simulink model "adaptive_joint_space_control"  (R2024b)
settings: Solver=VariableStepAuto  StartTime=0.0  StopTime=24*5  RelTol=1e-3
undefined symbols (not defined in the file): DiscIntNeverNeededParam, K_pi, Kd_c_ad, lambda, ml, pi0, q0, Tc
settings Model: Creator=storm  LastModifiedBy=giaco
settings OptimizationCC: ReuseModelBlockBuffer=off
settings DebuggingCC: UnconnectedInputMsg=warning  UnconnectedOutputMsg=warning  UnconnectedLineMsg=warning
settings ModelReferenceCC: EnableRefExpFcnMdlSchedulingChecks=on
settings RTWCC: GPUComputeCapability=3.5  DLArmComputeVersion=19.05

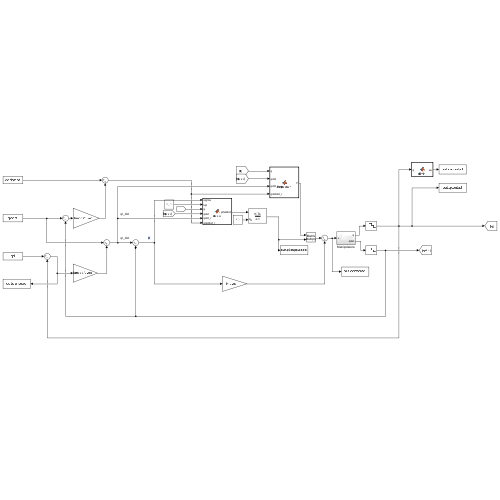
[thumbnail: Simulink's stored preview of the top-level diagram]
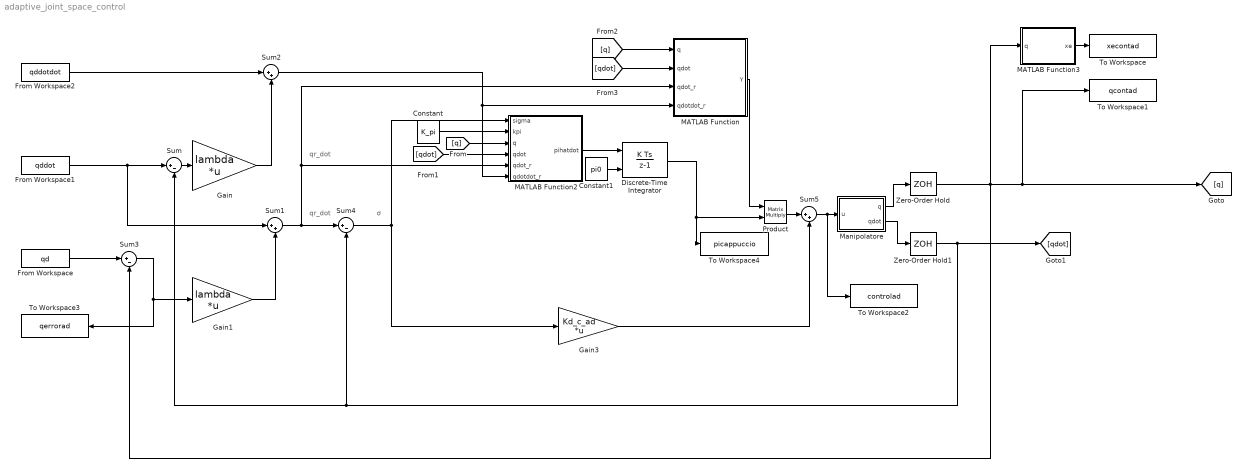
== system adaptive_joint_space_control ==
  note: σ
  note: qr_dot
  note: qr_dot
  Constant : Constant  Value=K_pi
  Constant1 : Constant  Value=pi0
  Discrete-Time Integrator : DiscreteIntegrator  InitialConditionSource=external  SampleTime=Tc  ICPrevOutput=DiscIntNeverNeededParam  ICPrevScaledInput=DiscIntNeverNeededParam
  From Workspace : FromWorkspace  VariableName=qd  SampleTime=Tc
  From Workspace1 : FromWorkspace  VariableName=qddot  SampleTime=Tc
  From Workspace2 : FromWorkspace  VariableName=qddotdot  SampleTime=Tc
  Gain : Gain  Gain=lambda  Multiplication=Matrix(K*u) (u vector)
  Gain1 : Gain  Gain=lambda  Multiplication=Matrix(K*u) (u vector)
  Gain3 : Gain  Gain=Kd_c_ad  Multiplication=Matrix(K*u) (u vector)
  MATLAB Function : MATLAB Function  TreatAsAtomicUnit=on
  MATLAB Function2 : MATLAB Function  TreatAsAtomicUnit=on
  MATLAB Function3 : MATLAB Function  TreatAsAtomicUnit=on
  Manipolatore : Subsystem
  Product : Product  Multiplication=Matrix(*)
  Sum : Sum  Inputs=|+-
  Sum1 : Sum  Inputs=|++
  Sum2 : Sum  Inputs=|++
  Sum3 : Sum  Inputs=|+-
  Sum4 : Sum  Inputs=|+-
  Sum5 : Sum  Inputs=|++
  To Workspace : ToWorkspace  VariableName=xecontad  SaveFormat=Structure With Time  SampleTime=-1
  To Workspace1 : ToWorkspace  VariableName=qcontad  SaveFormat=Structure With Time  SampleTime=-1
  To Workspace2 : ToWorkspace  VariableName=controlad  SaveFormat=Structure With Time  SampleTime=-1
  To Workspace3 : ToWorkspace  VariableName=qerrorad  SaveFormat=Structure With Time  SampleTime=-1
  To Workspace4 : ToWorkspace  VariableName=picappuccio  SaveFormat=Structure With Time  SampleTime=-1
  Zero-Order Hold : ZeroOrderHold  SampleTime=Tc
  Zero-Order Hold1 : ZeroOrderHold  SampleTime=Tc
  wires:
  MATLAB Function3/1(xe) -> To Workspace/1
  Zero-Order Hold/1 -> [q], To Workspace1/1, MATLAB Function3/1(q), Sum3/2
  Sum/1 -> Gain/1
  Gain/1 -> Sum2/2
  Gain1/1 -> Sum1/2
  Sum1/1 -> MATLAB Function2/5(qdot_r), MATLAB Function/3(qdot_r), Sum4/1
  Manipolatore/2(qdot) -> Zero-Order Hold1/1
  Zero-Order Hold1/1 -> [qdot], Sum/2, Sum4/2
  Manipolatore/1(q) -> Zero-Order Hold/1
  Sum4/1 -> MATLAB Function2/1(sigma), Gain3/1
  Gain3/1 -> Sum5/2
  Sum5/1 -> To Workspace2/1, Manipolatore/1(u)
  Sum2/1 -> MATLAB Function2/6(qdotdot_r), MATLAB Function/4(qdotdot_r)
  Constant/1 -> MATLAB Function2/2(kpi)
  [q] -> MATLAB Function2/3(q)
  [qdot] -> MATLAB Function2/4(qdot)
  MATLAB Function2/1(pihatdot) -> Discrete-Time Integrator/1
  Constant1/1 -> Discrete-Time Integrator/2
  MATLAB Function/1(Y) -> Product/1
  Discrete-Time Integrator/1 -> Product/2, To Workspace4/1
  Product/1 -> Sum5/1
  [qdot] -> MATLAB Function/2(qdot)
  [q] -> MATLAB Function/1(q)
  Sum3/1 -> To Workspace3/1, Gain1/1
  From Workspace/1 -> Sum3/1
  From Workspace1/1 -> Sum1/1, Sum/1
  From Workspace2/1 -> Sum2/1

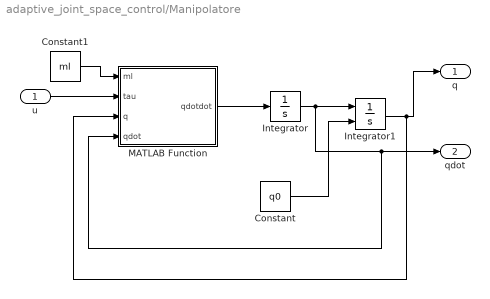
== system adaptive_joint_space_control/Manipolatore ==
  u : Inport
  Constant : Constant  Value=q0
  Constant1 : Constant  Value=ml
  Integrator : Integrator  InitialCondition=[0 0 0 0]'
  Integrator1 : Integrator  InitialConditionSource=external
  MATLAB Function : MATLAB Function  TreatAsAtomicUnit=on
  q : Outport
  qdot : Outport  Port=2
  wires:
  u/1 -> MATLAB Function/2(tau)
  MATLAB Function/1(qdotdot) -> Integrator/1
  Integrator/1 -> MATLAB Function/4(qdot), qdot/1, Integrator1/1
  Constant/1 -> Integrator1/2
  Integrator1/1 -> MATLAB Function/3(q), q/1
  Constant1/1 -> MATLAB Function/1(ml)

== matlab function adaptive_joint_space_control/MATLAB Function ==
  data: q input; Y output; qdot input; qdot_r input; qdotdot_r input
function Y = regressor(q,qdot,qdot_r,qdotdot_r)
% The 15 columns correspond to the parameters estimated by the controller.
a1=0.5;
a2=0.5;
l1=0.25;
l2=0.25;
ml1=20;
ml2=20;
ml3=10;
Il1=4;
Il2=4;
Il4=1;
kr1=1;
kr2=1;
kr3=50;
kr4=20;
Im1=0.01;
Im2=0.01;
Im3=0.005;
Im4=0.001;

Fm1=0.00005;
Fm2=0.00005;
Fm3=0.01;
Fm4=0.005;

Y=zeros(4,15);

Y=[l1^2*qdotdot_r(1),qdotdot_r(1),kr1^2*qdotdot_r(1),kr1^2*qdot_r(1),qdotdot_r(1)*(a1^2+l2^2+2*a1*l2*cos(q(2)))+qdotdot_r(2)*(l2^2+a1*l2*cos(q(2)))-a1*l2*sin(q(2))*qdot(2)*qdot_r(1)-a1*l2*sin(q(2))*qdot(1)*qdot_r(2)-a1*l2*sin(q(2))*qdot(2)*qdot_r(2) ,qdotdot_r(1)+qdotdot_r(2),qdotdot_r(1)+kr2*qdotdot_r(2),0,qdotdot_r(1)*(a1^2+a2^2+2*a1*a2*cos(q(2)))+qdotdot_r(2)*(a2^2+a1*a2*cos(q(2)))-a1*a2*sin(q(2))*qdot(2)*qdot_r(1)-a1*a2*sin(q(2))*qdot(1)*qdot_r(2)-a1*a2*sin(q(2))*qdot(2)*qdot_r(2),qdotdot_r(1)+qdotdot_r(2)+kr3*qdotdot_r(3),0,qdotdot_r(1)*(a1^2+a2^2+2*a1*a2*cos(q(2)))+qdotdot_r(2)*(a2^2+a1*a2*cos(q(2)))-a1*a2*sin(q(2))*qdot(2)*qdot_r(1)-a1*a2*sin(q(2))*qdot(1)*qdot_r(2)-a1*a2*sin(q(2))*qdot(2)*qdot_r(2),qdotdot_r(1)+qdotdot_r(2)+qdotdot_r(4),qdotdot_r(1)+qdotdot_r(2)+kr4*qdotdot_r(4),0;...
    0,0,0,0,qdotdot_r(1)*(l2^2+a1*l2*cos(q(2)))+qdotdot_r(2)*l2^2+a1*l2*sin(q(2))*qdot(1)*qdot_r(1),qdotdot_r(1)+qdotdot_r(2),kr2*qdotdot_r(1)+kr2^2*qdotdot_r(2),kr2^2*qdot_r(2),qdotdot_r(1)*(a2^2+a1*a2*cos(q(2)))+qdotdot_r(2)*a2^2+a1*a2*sin(q(2))*qdot(1)*qdot_r(1),qdotdot_r(1)+qdotdot_r(2)+kr3*qdotdot_r(3),0,qdotdot_r(1)*(a2^2+a1*a2*cos(q(2)))+qdotdot_r(2)*a2^2+a1*a2*sin(q(2))*qdot(1)*qdot_r(1),qdotdot_r(1)+qdotdot_r(2)+qdotdot_r(4),qdotdot_r(1)+qdotdot_r(2)+kr4*qdotdot_r(4),0;...
    0,0,0,0,0,0,0,0,qdotdot_r(3)+9.81,kr3*qdotdot_r(1)+kr3*qdotdot_r(2)+kr3^2*qdotdot_r(3),kr3^2*qdot_r(3),qdotdot_r(3)+9.81,0,0,0;...
    0,0,0,0,0,0,0,0,0,0,0,0,qdotdot_r(1)+qdotdot_r(2)+qdotdot_r(4),kr4*qdotdot_r(1)+kr4*qdotdot_r(2)+kr4^2*qdotdot_r(4),kr4^2*qdot_r(4)];
end

== matlab function adaptive_joint_space_control/MATLAB Function2 ==
  data: sigma input; pihatdot output; kpi input; q input; qdot input; qdot_r input; qdotdot_r input
function pihatdot = adatt(sigma,kpi,q,qdot,qdot_r,qdotdot_r)
% Weight the update by the inverse adaptation gain.

a1=0.5;
a2=0.5;
l1=0.25;
l2=0.25;
ml1=20;
ml2=20;
ml3=10;
Il1=4;
Il2=4;
Il4=1;
kr1=1;
kr2=1;
kr3=50;
kr4=20;
Im1=0.01;
Im2=0.01;
Im3=0.005;
Im4=0.001;

Fm1=0.00005;
Fm2=0.00005;
Fm3=0.01;
Fm4=0.005;

Y=[l1^2*qdotdot_r(1),qdotdot_r(1),kr1^2*qdotdot_r(1),kr1^2*qdot_r(1),qdotdot_r(1)*(a1^2+l2^2+2*a1*l2*cos(q(2)))+qdotdot_r(2)*(l2^2+a1*l2*cos(q(2)))-a1*l2*sin(q(2))*qdot(2)*qdot_r(1)-a1*l2*sin(q(2))*qdot(1)*qdot_r(2)-a1*l2*sin(q(2))*qdot(2)*qdot_r(2) ,qdotdot_r(1)+qdotdot_r(2),qdotdot_r(1)+kr2*qdotdot_r(2),0,qdotdot_r(1)*(a1^2+a2^2+2*a1*a2*cos(q(2)))+qdotdot_r(2)*(a2^2+a1*a2*cos(q(2)))-a1*a2*sin(q(2))*qdot(2)*qdot_r(1)-a1*a2*sin(q(2))*qdot(1)*qdot_r(2)-a1*a2*sin(q(2))*qdot(2)*qdot_r(2),qdotdot_r(1)+qdotdot_r(2)+kr3*qdotdot_r(3),0,qdotdot_r(1)*(a1^2+a2^2+2*a1*a2*cos(q(2)))+qdotdot_r(2)*(a2^2+a1*a2*cos(q(2)))-a1*a2*sin(q(2))*qdot(2)*qdot_r(1)-a1*a2*sin(q(2))*qdot(1)*qdot_r(2)-a1*a2*sin(q(2))*qdot(2)*qdot_r(2),qdotdot_r(1)+qdotdot_r(2)+qdotdot_r(4),qdotdot_r(1)+qdotdot_r(2)+kr4*qdotdot_r(4),0;...
    0,0,0,0,qdotdot_r(1)*(l2^2+a1*l2*cos(q(2)))+qdotdot_r(2)*l2^2+a1*l2*sin(q(2))*qdot(1)*qdot_r(1),qdotdot_r(1)+qdotdot_r(2),kr2*qdotdot_r(1)+kr2^2*qdotdot_r(2),kr2^2*qdot_r(2),qdotdot_r(1)*(a2^2+a1*a2*cos(q(2)))+qdotdot_r(2)*a2^2+a1*a2*sin(q(2))*qdot(1)*qdot_r(1),qdotdot_r(1)+qdotdot_r(2)+kr3*qdotdot_r(3),0,qdotdot_r(1)*(a2^2+a1*a2*cos(q(2)))+qdotdot_r(2)*a2^2+a1*a2*sin(q(2))*qdot(1)*qdot_r(1),qdotdot_r(1)+qdotdot_r(2)+qdotdot_r(4),qdotdot_r(1)+qdotdot_r(2)+kr4*qdotdot_r(4),0;...
    0,0,0,0,0,0,0,0,qdotdot_r(3)+9.81,kr3*qdotdot_r(1)+kr3*qdotdot_r(2)+kr3^2*qdotdot_r(3),kr3^2*qdot_r(3),qdotdot_r(3)+9.81,0,0,0;...
    0,0,0,0,0,0,0,0,0,0,0,0,qdotdot_r(1)+qdotdot_r(2)+qdotdot_r(4),kr4*qdotdot_r(1)+kr4*qdotdot_r(2)+kr4^2*qdotdot_r(4),kr4^2*qdot_r(4)];

pihatdot=inv(kpi)*Y'*sigma;

end

== matlab function adaptive_joint_space_control/Manipolatore/MATLAB Function ==
  data: ml input; qdotdot output; tau input; q input; qdot input
function qdotdot= Dinamica_diretta(ml,tau,q,qdot)
% Plant dynamics: subtract Coriolis, friction, and gravity before solving for acceleration.
a1=0.5;
a2=0.5;
l1=0.25;
l2=0.25;
ml1=20;
ml2=20;
ml3=10;
Il1=4;
Il2=4;
Il4=1;
kr1=1;
kr2=1;
kr3=50;
kr4=20;
Im1=0.01;
Im2=0.01;
Im3=0.005;
Im4=0.001;

Fm1=0.00005;
Fm2=0.00005;
Fm3=0.01;
Fm4=0.005;

mhe=4; % Payload mass parameter [kg]
% Link and rotor Jacobians used to assemble the inertia matrix.
Jpl1=[-l1*sin(q(1)) 0 0 0;
    l1*cos(q(1)) 0 0 0;
    0 0 0 0];

Jpl2=[-a1*sin(q(1))-l2*sin(q(1)+q(2)),-l2*sin(q(1)+q(2)),0,0;
    a1*cos(q(1))+l2*cos(q(1)+q(2)),l2*cos(q(1)+q(2)),0,0;
    0,0,0,0];

Jpl4=[-a1*sin(q(1))-a2*sin(q(1)+q(2)),-a2*sin(q(1)+q(2)),0,0;
    a1*cos(q(1))+a2*cos(q(1)+q(2)),a2*cos(q(1)+q(2)),0,0;
    0,0,1,0];

Jol1=[zeros(2,4);
    1 0 0 0];

Jol2=[zeros(2,4);
    1 1 0 0];

Jol4=[zeros(2,4);
    1 1 0 1];

Jom1=[zeros(2,4);
    kr1 0 0 0];

Jom2=[zeros(2,4);
    1 kr2 0 0];

Jom3=[zeros(2,4);
    1 1 kr3 0];

Jom4=[zeros(2,4);
    1 1 0 kr4];

B=ml1*(Jpl1'*Jpl1)+Jol1'*Il1*Jol1+Jom1'*Im1*Jom1...
    +ml2*(Jpl2'*Jpl2)+Jol2'*Il2*Jol2+Jom2'*Im2*Jom2...
    +Jom3'*Im3*Jom3...
    +(ml+ml3)*(Jpl4'*Jpl4)+Jol4'*Il4*Jol4+Jom4'*Im4*Jom4;

c=zeros(4,4,4);

Jpl1dq1=[-l1*cos(q(1)) 0 0 0;
    -l1*sin(q(1)) 0 0 0;
    0 0 0 0];

Jpl1dq2=zeros(3,4);

Jpl2dq1=[-a1*cos(q(1))-l2*cos(q(1)+q(2)),-l2*cos(q(1)+q(2)),0,0;
    -a1*sin(q(1))-l2*sin(q(1)+q(2)),-l2*sin(q(1)+q(2)),0,0;
    0,0,0,0];

Jpl2dq2=[-l2*cos(q(1)+q(2)),-l2*cos(q(1)+q(2)),0,0;
    -l2*sin(q(1)+q(2)),-l2*sin(q(1)+q(2)),0,0;
    0,0,0,0];

Jpl4dq1=[-a1*cos(q(1))-a2*cos(q(1)+q(2)),-a2*cos(q(1)+q(2)),0,0;
    -a1*sin(q(1))-a2*sin(q(1)+q(2)),-a2*sin(q(1)+q(2)),0,0;
    0,0,0,0];

Jpl4dq2=[-a2*cos(q(1)+q(2)),-a2*cos(q(1)+q(2)),0,0;
    -a2*sin(q(1)+q(2)),-a2*sin(q(1)+q(2)),0,0;
    0,0,0,0];

dBdq1=ml1*(Jpl1dq1'*Jpl1+Jpl1'*Jpl1dq1)+ml2*(Jpl2dq1'*Jpl2+Jpl2'*Jpl2dq1)+ml3*(Jpl4dq1'*Jpl4+Jpl4'*Jpl4dq1);
dBdq2=ml1*(Jpl1dq2'*Jpl1+Jpl1'*Jpl1dq2)+ml2*(Jpl2dq2'*Jpl2+Jpl2'*Jpl2dq2)+ml3*(Jpl4dq2'*Jpl4+Jpl4'*Jpl4dq2);

c(1,1,2)=-ml2*a1*l2*sin(q(2))-ml3*a1*a2*sin(q(2));
c(1,2,2)=c(1,1,2);
c(2,1,1)=-c(1,1,2);

C=zeros(4,4);
    for i=1:4
        for j=1:4
            for k=1:4
                C(i,j)=c(i,j,k)*qdot(k);
            end
        end
    end

g=[0 0 9.81*(ml+ml3) 0]';

Fv=diag([kr1^2*Fm1,kr2^2*Fm2,kr3^2*Fm3,kr4^2*Fm4]);
qdotdot=inv(B)*(tau-C*qdot-Fv*qdot-g);
end

== matlab function adaptive_joint_space_control/MATLAB Function3 ==
  data: q input; xe output
function xe = dirkin(q)
% Pose in base coordinates, ordered as [x; y; z; phi].
a1=0.5;
a2=a1;
d0=1;

xe=[a1*cos(q(1))+a2*cos(q(1)+q(2));...
    a1*sin(q(1))+a2*sin(q(1)+q(2));...
    d0+q(3);...
    q(1)+q(2)+q(4)];
end
